simulink model "heli_q8"  (R2020b)
settings: Solver=ode1  StartTime=0.0  StopTime=inf  FixedStep=0.002  RelTol=1e-3  EnableMultiTasking=on
PostLoadFcn:
  | qc_set_target_type(getConfigSet(bdroot, 'QUARC Default Target Configuration'));
values from neighbouring files (symbols this model uses):
  elevation_offset = 0.5    [init_heli.m]
  F = [K(1,1) K(1,3) ... (first row only)    [init_heli.m]
  Joystick_gain_x = 2    [init_heli.m]
  Joystick_gain_y = -0.5    [init_heli.m]
  K = lqr(A, B, Q, R)    [init_heli.m]
undefined symbols (not defined in the file or in its folder): HIL, qc_get_step_size
libraries: quarc_library x4, simulink x4, cstblocks x2
settings Model: SimulationMode=external  ExtModeTrigDuration=6000  Creator=Rchan  LastModifiedBy=oscarlb
settings SolverCC: PositivePriorityOrder=on
settings DataIOCC: LimitDataPoints=on  SaveFormat=Array  SignalLoggingSaveFormat=ModelDataLogs  ReturnWorkspaceOutputs=off
settings OptimizationCC: ExpressionDepthLimit=2147483647  InitFltsAndDblsToZero=on  LifeSpan=inf
settings DebuggingCC: SaveWithParameterizedLinksMsg=none  UnderspecifiedInitializationDetection=Classic  MergeDetectMultiDrivingBlocksExec=none  SolverPrmCheckMsg=warning  MultiTaskDSMMsg=warning  MultiTaskCondExecSysMsg=none  FcnCallInpInsideContextMsg=warning  AllowSymbolicDim=off  StateNameClashWarn=warning  SFUnexpectedBacktrackingDiag=warning  SFNoUnconditionalDefaultTransitionDiag=warning  SFExecutionAtInitializationDiag=none  ArithmeticOperatorsInVariantConditions=warning
settings HardwareCC: ProdBitPerPointer=32  ProdBitPerSizeT=32  ProdBitPerPtrDiffT=32  ProdLargestAtomicFloat=None  ProdIntDivRoundTo=Undefined  ProdEndianess=Unspecified  ProdWordSize=32  ProdHWDeviceType=32-bit Generic
settings ModelReferenceCC: PropagateSignalLabelsOutOfModel=off
settings SFSimCC: SimUseLocalCustomCode=off  CustomCodeUndefinedFunction=UseInterfaceOnly
settings RTWCC: Description=QUARC Win64 Target  SystemTargetFile=quarc_win64.tlc  TemplateMakefile=quarc_default_tmf  RTWUseLocalCustomCode=off
settings CodeAppCC: StateflowObjectComments=on
settings GRTTargetCC: TargetLangStandard=C89/C90 (ANSI)  ParMdlRefBuildCompliant=off  CompOptLevelCompliant=off  CombineOutputUpdateFcns=off  MatFileLogging=off  GRTInterface=on  UseToolchainInfoCompliant=off  ExtMode=on  ExtModeMexFile=quarc_comm
settings ConfigComp: CovMetricSettings=dw  CovSaveCumulativeToWorkspaceVar=on  CovSaveSingleToWorkspaceVar=on  CovExternalEMLEnable=off  CovSFcnEnable=off

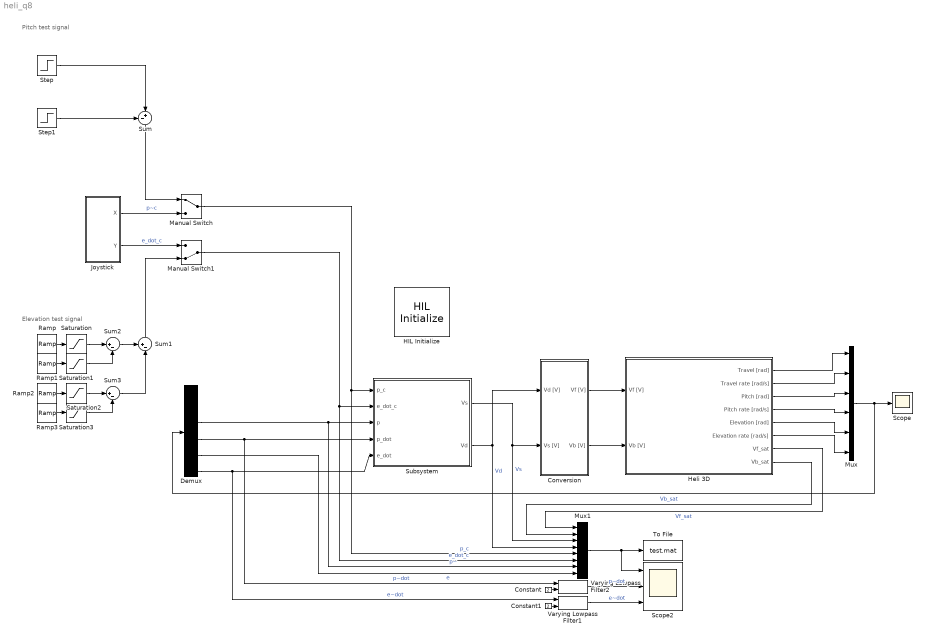
== system heli_q8 ==
  note: Pitch test signal
  note: Elevation test signal
  Constant : Constant  Value=2
  Constant1 : Constant  Value=2
  Conversion : Subsystem
  Demux : Demux  Outputs=6
  HIL Initialize : quarc_library/Data Acquisition/Generic/Configuration/HIL Initialize  Priority=-99  object_name=HIL-1  board_type=q8_usb  board_number=0  board_options=update_rate=normal;decimation=1  exclusive=off  active=off  hardware_clocks=[0:2]  clock_modes=[]  initial_clock_frequencies=[]  set_clock_params_at_start=off  set_clock_params_at_switch_in=off  set_clock_frequencies_at_start=off  set_clock_frequencies_at_switch_in=off  analog_input_channels=[0:7]  analog_input_configurations=[]  analog_input_maximums=10  analog_input_minimums=-10  set_analog_input_params_at_start=on  set_analog_input_params_at_switch_in=off  analog_output_channels=[0:7]  analog_output_maximums=10  analog_output_minimums=-10  initial_analog_outputs=[0]  final_analog_outputs=[0]  watchdog_analog_outputs=0  set_analog_output_params_at_start=on  set_analog_output_params_at_switch_in=off  set_analog_outputs_at_start=on  set_analog_outputs_at_switch_in=off  set_analog_outputs_at_terminate=on  set_analog_outputs_at_switch_out=off  set_analog_outputs_on_watchdog=off  digital_input_channels=[]  digital_output_channels=[]  digital_output_configuration=[]  initial_digital_outputs=[1]  final_digital_outputs=[1]  watchdog_digital_outputs=[1]  set_digital_output_params_at_start=off  set_digital_output_params_at_switch_in=off  set_digital_outputs_at_start=on  set_digital_outputs_at_switch_in=off  set_digital_outputs_at_terminate=on  set_digital_outputs_at_switch_out=off  set_digital_outputs_on_watchdog=off  encoder_channels=[0:7]  quadrature=[4]  encoder_filter_frequency=[]  initial_encoder_counts=[0]  set_encoder_params_at_start=on  set_encoder_params_at_switch_in=off  set_encoder_counts_at_start=on  set_encoder_counts_at_switch_in=off  pwm_channels=[0:7]  pwm_modes=0  pwm_frequency=99.532799999999995e6/4095  pwm_configuration=[0]  pwm_alignment=[0]  pwm_polarity=[1]  pwm_leading_deadband=[0]  pwm_trailing_deadband=[0]  initial_pwm_outputs=[0]  final_pwm_outputs=[0]  watchdog_pwm_outputs=[0]  set_pwm_params_at_start=on  set_pwm_params_at_switch_in=off  set_pwm_outputs_at_start=on  set_pwm_outputs_at_switch_in=off  set_pwm_outputs_at_terminate=on  set_pwm_outputs_at_switch_out=off  set_pwm_outputs_on_watchdog=off  other_output_channels=[]  initial_other_outputs=[]  final_other_outputs=[]  watchdog_other_outputs=[]  set_other_outputs_at_start=off  set_other_outputs_at_switch_in=off  set_other_outputs_at_terminate=off  set_other_outputs_at_switch_out=off  set_other_outputs_on_watchdog=off
  Heli 3D : Subsystem
  Joystick : Subsystem
  Manual Switch : ManualSwitch
  Manual Switch1 : ManualSwitch  CurrentSetting=0
  Mux : Mux  Inputs=6
  Mux1 : Mux  Inputs=8
  Ramp : simulink/Sources/Ramp  slope=0.03  start=0  InitialOutput=0
  Ramp1 : simulink/Sources/Ramp  slope=0.03  start=5  InitialOutput=0
  Ramp2 : simulink/Sources/Ramp  slope=0.03  start=45  InitialOutput=0
  Ramp3 : simulink/Sources/Ramp  slope=0.03  start=50  InitialOutput=0
  Saturation : Saturate  UpperLimit=0.15  LowerLimit=0
  Saturation1 : Saturate  UpperLimit=0.15  LowerLimit=0
  Saturation2 : Saturate  UpperLimit=0.15  LowerLimit=0
  Saturation3 : Saturate  UpperLimit=0.13  LowerLimit=0
  Scope : Scope
  Scope2 : Scope  NumInputPorts=3
  Step : Step  Time=10  After=pi/8  SampleTime=0
  Step1 : Step  Time=40  After=pi/8  SampleTime=0
  Subsystem : Subsystem
  Sum : Sum  Inputs=-+|
  Sum1 : Sum  Inputs=+-|
  Sum2 : Sum  Inputs=|+-
  Sum3 : Sum  Inputs=|+-
  To File : ToFile  Filename=test.mat
  Varying Lowpass Filter1 : cstblocks/Linear Parameter Varying/Varying Lowpass Filter  N=1
  Varying Lowpass Filter2 : cstblocks/Linear Parameter Varying/Varying Lowpass Filter  N=1
  wires:
  Conversion/2(Vb [V]) -> Heli 3D/2(Vb [V])
  Conversion/1(Vf [V]) -> Heli 3D/1(Vf [V])
  Heli 3D/1(Travel [rad]) -> Mux/1
  Heli 3D/2(Travel rate [rad/s]) -> Mux/2
  Heli 3D/3(Pitch [rad]) -> Mux/3
  Heli 3D/4(Pitch rate [rad/s]) -> Mux/4
  Heli 3D/5(Elevation [rad]) -> Mux/5
  Heli 3D/6(Elevation rate [rad/s]) -> Mux/6
  Mux/1 -> Demux/1, Scope/1
  Mux1/1 -> Scope2/1, To File/1
  Subsystem/2(Vd) -> Mux1/4, Conversion/1(Vd [V])  "Vd"
  Demux/3 -> Mux1/7, Subsystem/3(p)  "p~"
  Demux/4 -> Varying Lowpass Filter2/1, Subsystem/4(p_dot)  "p~dot"
  Demux/6 -> Varying Lowpass Filter1/1, Subsystem/5(e_dot)  "e~dot"
  Manual Switch/1 -> Mux1/5, Subsystem/1(p_c)  "p_c"
  Manual Switch1/1 -> Mux1/6, Subsystem/2(e_dot_c)  "e_dot_c"
  Joystick/2(Y) -> Manual Switch1/1  "e_dot_c"
  Joystick/1(X) -> Manual Switch/2  "p~c"
  Subsystem/1(Vs) -> Conversion/2(Vs [V]), Mux1/3  "Vs"
  Constant1/1 -> Varying Lowpass Filter1/2
  Constant/1 -> Varying Lowpass Filter2/2
  Demux/5 -> Mux1/8  "e"
  Varying Lowpass Filter2/1 -> Scope2/2  "p~dot"
  Varying Lowpass Filter1/1 -> Scope2/3  "e~dot"
  Sum/1 -> Manual Switch/1
  Step/1 -> Sum/2
  Step1/1 -> Sum/1
  Sum1/1 -> Manual Switch1/2
  Ramp/1 -> Saturation/1
  Saturation/1 -> Sum2/1
  Sum2/1 -> Sum1/1
  Ramp1/1 -> Saturation1/1
  Saturation1/1 -> Sum2/2
  Saturation3/1 -> Sum3/2
  Ramp3/1 -> Saturation3/1
  Saturation2/1 -> Sum3/1
  Ramp2/1 -> Saturation2/1
  Sum3/1 -> Sum1/2
  Heli 3D/8(Vb_sat) -> Mux1/2  "Vb_sat"
  Heli 3D/7(Vf_sat) -> Mux1/1  "Vf_sat"

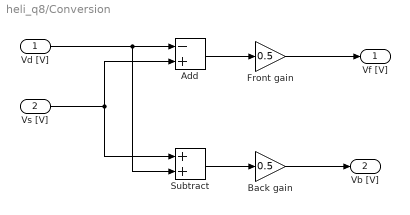
== system heli_q8/Conversion ==
  Vd [V] : Inport
  Vs [V] : Inport  Port=2
  Add : Sum  Inputs=-+
  Back gain : Gain  Gain=0.5
  Front gain : Gain  Gain=0.5
  Subtract : Sum
  Vf [V] : Outport
  Vb [V] : Outport  Port=2
  wires:
  Vd [V]/1 -> Subtract/2, Add/1
  Vs [V]/1 -> Subtract/1, Add/2
  Subtract/1 -> Back gain/1
  Back gain/1 -> Vb [V]/1
  Add/1 -> Front gain/1
  Front gain/1 -> Vf [V]/1

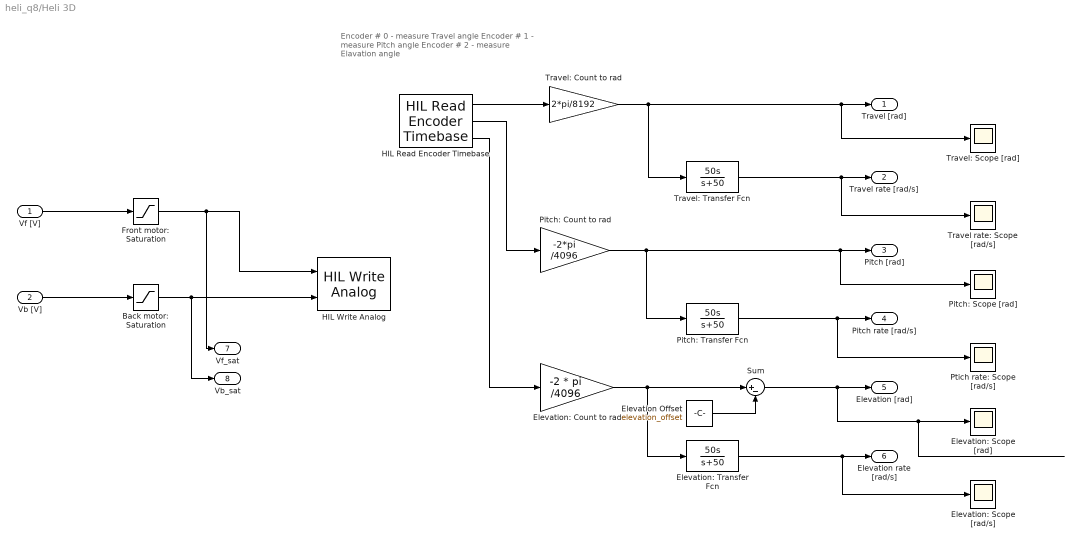
== system heli_q8/Heli 3D ==
  note: Encoder # 0 - measure Travel angle
      | Encoder # 1 - measure Pitch angle
      | Encoder # 2 - measure Elavation angle
  Vf [V] : Inport
  Vb [V] : Inport  Port=2
  Back motor: Saturation : Saturate  UpperLimit=5  LowerLimit=-5
  Elevation Offset : Constant  Value=elevation_offset
  Elevation: Count to rad : Gain  Gain=-2 * pi /4096
  Elevation: Scope [rad/s] : Scope
  Elevation: Scope [rad] : Scope
  Elevation: Transfer Fcn : TransferFcn  Numerator=[50 0]  Denominator=[1 50]
  Front motor: Saturation : Saturate  UpperLimit=5  LowerLimit=-5
  HIL Read Encoder Timebase : quarc_library/Data Acquisition/Generic/Timebases/HIL Read Encoder Timebase  object_name=HIL-1  clock=0  channels=[0:2]  active=on  vector_output=off  data_type_mode=Inherit via back propagation  data_type=double  overflow_mode=Error on overflow  samples_in_buffer=max(ceil(1/qc_get_step_size), 1)
  HIL Write Analog : quarc_library/Data Acquisition/Generic/Immediate I//O/HIL Write Analog  object_name=HIL-1  channels=[0:1]  sample_time=-1  active=off  vector_input=off
  Pitch: Count to rad : Gain  Gain=-2*pi /4096
  Pitch: Scope [rad] : Scope
  Pitch: Transfer Fcn : TransferFcn  Numerator=[50 0]  Denominator=[1 50]
  Ptich rate: Scope [rad/s] : Scope
  Sum : Sum  Inputs=|+-
  Travel rate: Scope [rad/s] : Scope
  Travel: Count to rad : Gain  Gain=2*pi/8192
  Travel: Scope [rad] : Scope
  Travel: Transfer Fcn : TransferFcn  Numerator=[50 0]  Denominator=[1 50]
  Travel [rad] : Outport
  Travel rate [rad/s] : Outport  Port=2
  Pitch [rad] : Outport  Port=3
  Pitch rate [rad/s] : Outport  Port=4
  Elevation [rad] : Outport  Port=5
  Elevation rate [rad/s] : Outport  Port=6
  Vf_sat : Outport  Port=7
  Vb_sat : Outport  Port=8
  wires:
  HIL Read Encoder Timebase/1 -> Travel: Count to rad/1
  HIL Read Encoder Timebase/2 -> Pitch: Count to rad/1
  HIL Read Encoder Timebase/3 -> Elevation: Count to rad/1
  Travel: Count to rad/1 -> Travel: Scope [rad]/1, Travel [rad]/1, Travel: Transfer Fcn/1
  Travel: Transfer Fcn/1 -> Travel rate: Scope [rad/s]/1, Travel rate [rad/s]/1
  Pitch: Count to rad/1 -> Pitch: Transfer Fcn/1, Pitch: Scope [rad]/1, Pitch [rad]/1
  Pitch: Transfer Fcn/1 -> Ptich rate: Scope [rad/s]/1, Pitch rate [rad/s]/1
  Elevation: Count to rad/1 -> Sum/1, Elevation: Transfer Fcn/1
  Elevation: Transfer Fcn/1 -> Elevation: Scope [rad/s]/1, Elevation rate [rad/s]/1
  Vf [V]/1 -> Front motor: Saturation/1
  Vb [V]/1 -> Back motor: Saturation/1
  Front motor: Saturation/1 -> Vf_sat/1, HIL Write Analog/1
  Back motor: Saturation/1 -> Vb_sat/1, HIL Write Analog/2
  Sum/1 -> Elevation: Scope [rad]/1, Elevation [rad]/1
  Elevation Offset/1 -> Sum/2

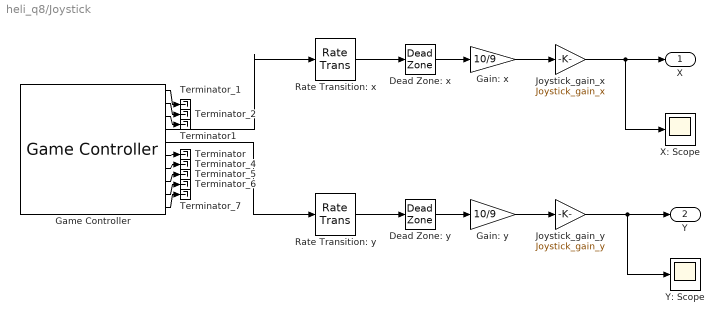
== system heli_q8/Joystick ==
  Dead Zone: x : DeadZone  LowerValue=-0.1  UpperValue=0.1  SaturateOnIntegerOverflow=on
  Dead Zone: y : DeadZone  LowerValue=-0.1  UpperValue=0.1  SaturateOnIntegerOverflow=on
  Gain: x : Gain  Gain=10/9
  Gain: y : Gain  Gain=10/9
  Game Controller : quarc_library/Devices/Peripherals/Target/Game Controller  controller=1  buffer_size=12  deadzone=[]  saturation=[]  sample_time=max(qc_get_step_size, 0.01)  auto_center=off  enabled=on
      settings: SourceProductName=QUARC Targets
  Joystick_gain_x : Gain  Gain=Joystick_gain_x
  Joystick_gain_y : Gain  Gain=Joystick_gain_y
  Rate Transition: x : RateTransition
  Rate Transition: y : RateTransition
  Terminator : Terminator
  Terminator1 : Terminator
  Terminator_{1..2,4..7} (6 alike) : Terminator
  X: Scope : Scope
  Y: Scope : Scope
  X : Outport
  Y : Outport  Port=2
  wires:
  Rate Transition: y/1 -> Dead Zone: y/1
  Rate Transition: x/1 -> Dead Zone: x/1
  Game Controller/5 -> Rate Transition: y/1
  Game Controller/4 -> Rate Transition: x/1
  Game Controller/1 -> Terminator_1/1
  Game Controller/2 -> Terminator_2/1
  Game Controller/7 -> Terminator_4/1
  Game Controller/8 -> Terminator_5/1
  Game Controller/9 -> Terminator_6/1
  Game Controller/10 -> Terminator_7/1
  Game Controller/3 -> Terminator1/1
  Game Controller/6 -> Terminator/1
  Dead Zone: x/1 -> Gain: x/1
  Dead Zone: y/1 -> Gain: y/1
  Gain: x/1 -> Joystick_gain_x/1
  Gain: y/1 -> Joystick_gain_y/1
  Joystick_gain_x/1 -> X/1, X: Scope/1
  Joystick_gain_y/1 -> Y: Scope/1, Y/1

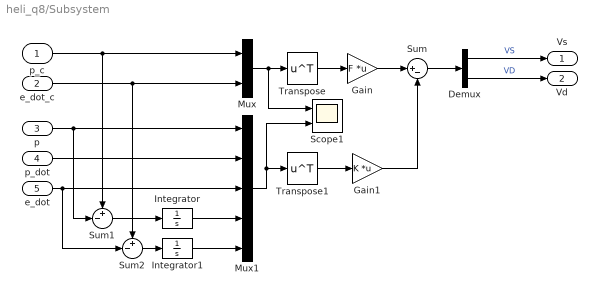
== system heli_q8/Subsystem ==
  p_c : Inport
  e_dot_c : Inport  Port=2
  p : Inport  Port=3
  p_dot : Inport  Port=4
  e_dot : Inport  Port=5
  Demux : Demux  Outputs=2
  Gain : Gain  Gain=F  Multiplication=Matrix(K*u) (u vector)
  Gain1 : Gain  Gain=K  Multiplication=Matrix(K*u) (u vector)
  Integrator : Integrator
  Integrator1 : Integrator
  Mux : Mux  Inputs=2
  Mux1 : Mux  Inputs=5
  Scope1 : Scope  NumInputPorts=2
  Sum : Sum  Inputs=|+-
  Sum1 : Sum  Inputs=+-|
  Sum2 : Sum  Inputs=+-|
  Transpose : Math  Operator=transpose  SaturateOnIntegerOverflow=on
  Transpose1 : Math  Operator=transpose  SaturateOnIntegerOverflow=on
  Vs : Outport
  Vd : Outport  Port=2
  wires:
  p_c/1 -> Sum1/1, Mux/1
  p/1 -> Sum1/2, Mux1/1
  p_dot/1 -> Mux1/2
  e_dot/1 -> Sum2/2, Mux1/3
  Mux/1 -> Scope1/1, Transpose/1
  Mux1/1 -> Scope1/2, Transpose1/1
  Gain/1 -> Sum/1
  Gain1/1 -> Sum/2
  Transpose/1 -> Gain/1
  Transpose1/1 -> Gain1/1
  Sum/1 -> Demux/1
  Demux/1 -> Vs/1  "VS"
  e_dot_c/1 -> Mux/2, Sum2/1
  Demux/2 -> Vd/1  "VD"
  Sum1/1 -> Integrator/1
  Sum2/1 -> Integrator1/1
  Integrator/1 -> Mux1/4
  Integrator1/1 -> Mux1/5
